simulink model "pmsm_foc"  (R2026a)
settings: Solver=ode4  StopTime=t_stop  FixedStep=P.Tsim
undefined symbols (not defined in the file or in its folder): P
settings Model: Creator=mask9  LastModifiedBy=mask9

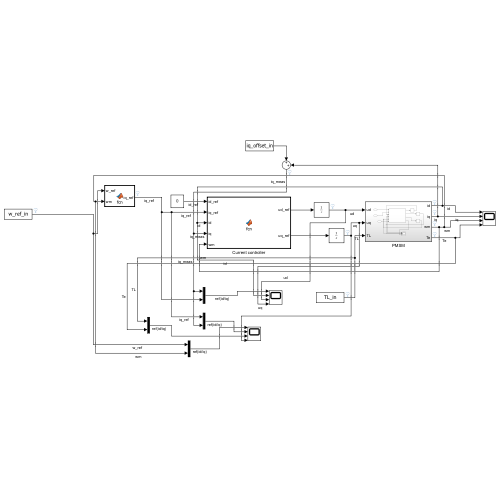
[thumbnail: Simulink's stored preview of the top-level diagram]
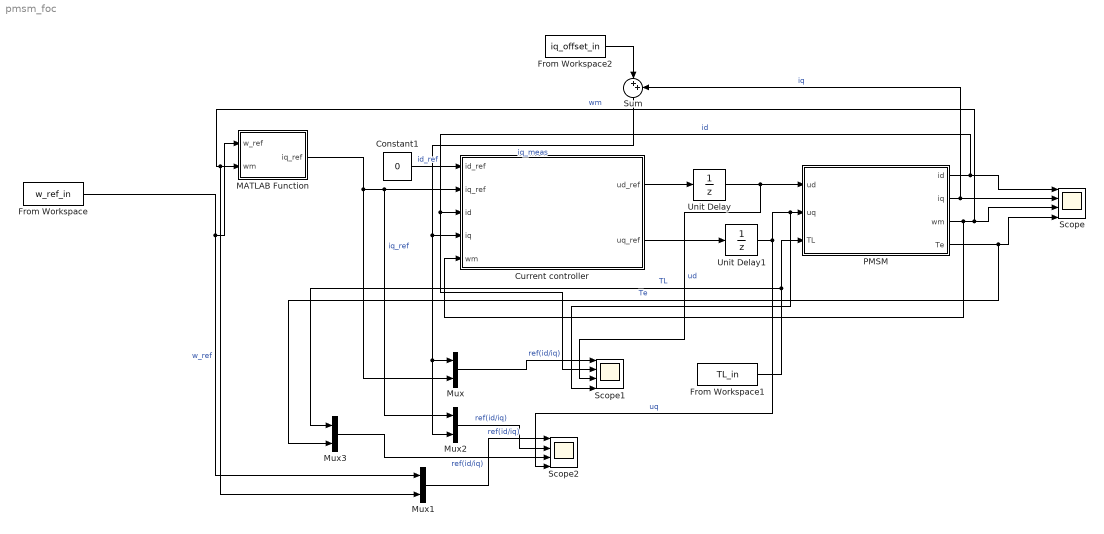
== system pmsm_foc ==
  Constant1 : Constant  Value=0
  Current controller : MATLAB Function  TreatAsAtomicUnit=on
  From Workspace : FromWorkspace  VariableName=w_ref_in  OutputAfterFinalValue=Holding final value
  From Workspace1 : FromWorkspace  VariableName=TL_in  OutputAfterFinalValue=Holding final value
  From Workspace2 : FromWorkspace  VariableName=iq_offset_in  OutputAfterFinalValue=Holding final value
  MATLAB Function : MATLAB Function  TreatAsAtomicUnit=on
  Mux{,1..3} (4 alike) : Mux  Inputs=2
  PMSM : Subsystem
  Scope : Scope  NumInputPorts=4
      settings: ActiveDisplayYMinimum=-7.6366046991371559E-6  ActiveDisplayYMaximum=6.8729442292234425E-5
  Scope1 : Scope  NumInputPorts=4
      settings: ActiveDisplayYMinimum=-60.523528989207882  ActiveDisplayYMaximum=544.71176090287111
  Scope2 : Scope  NumInputPorts=4
      settings: ActiveDisplayYMinimum=-6.2565775953438321  ActiveDisplayYMaximum=56.309198358094505  DataLoggingVariableName=ScopeData2
  Sum : Sum  Inputs=|++
  Unit Delay : UnitDelay  SampleTime=P.Ts
  Unit Delay1 : UnitDelay  SampleTime=P.Ts
  wires:
  From Workspace1/1 -> Mux3/1, PMSM/3(TL)  "TL"
  PMSM/1(id) -> Scope1/2, Current controller/3(id), Scope/1  "id"
  PMSM/2(iq) -> Sum/2, Scope/2  "iq"
  PMSM/3(wm) -> Current controller/5(wm), Mux1/2, MATLAB Function/2(wm), Scope/3  "wm"
  PMSM/4(Te) -> Mux3/2, Scope/4  "Te"
  Current controller/1(ud_ref) -> Unit Delay/1
  Unit Delay/1 -> Scope1/3, PMSM/1(ud)  "ud"
  Current controller/2(uq_ref) -> Unit Delay1/1
  Unit Delay1/1 -> Scope1/4, PMSM/2(uq), Scope2/4  "uq"
  Constant1/1 -> Current controller/1(id_ref)  "id_ref"
  Mux/1 -> Scope1/1  "ref(id/iq)"
  MATLAB Function/1(iq_ref) -> Mux/2, Mux2/1, Current controller/2(iq_ref)  "iq_ref"
  From Workspace/1 -> Mux1/1, MATLAB Function/1(w_ref)  "w_ref"
  Mux1/1 -> Scope2/1  "ref(id/iq)"
  Mux2/1 -> Scope2/2  "ref(id/iq)"
  Mux3/1 -> Scope2/3  "ref(id/iq)"
  From Workspace2/1 -> Sum/1
  Sum/1 -> Current controller/4(iq), Mux/1, Mux2/2  "iq_meas"

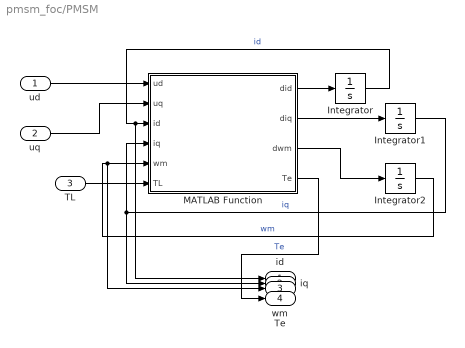
== system pmsm_foc/PMSM ==
  ud : Inport
  uq : Inport  Port=2
  TL : Inport  Port=3
  Integrator : Integrator
  Integrator1 : Integrator
  Integrator2 : Integrator
  MATLAB Function : MATLAB Function  TreatAsAtomicUnit=on
  id : Outport
  iq : Outport  Port=2
  wm : Outport  Port=3
  Te : Outport  Port=4
  wires:
  MATLAB Function/2(diq) -> Integrator1/1
  Integrator2/1 -> wm/1, MATLAB Function/5(wm)  "wm"
  MATLAB Function/3(dwm) -> Integrator2/1
  Integrator/1 -> id/1, MATLAB Function/3(id)  "id"
  uq/1 -> MATLAB Function/2(uq)
  Integrator1/1 -> iq/1, MATLAB Function/4(iq)  "iq"
  MATLAB Function/1(did) -> Integrator/1
  ud/1 -> MATLAB Function/1(ud)
  TL/1 -> MATLAB Function/6(TL)
  MATLAB Function/4(Te) -> Te/1  "Te"

== matlab function pmsm_foc/Current controller ==
  settings: updateMethod=DISCRETE  sampleTime=P.Ts
  data: id_ref input; ud_ref output; iq_ref input; id input; iq input; wm input; uq_ref output; P parameter
function [ud_ref, uq_ref] = fcn(id_ref, iq_ref, id, iq, wm, P)
persistent xd xq
if isempty(xd), xd = 0; xq = 0; end

we = P.p * wm;
ed = id_ref - id;
eq = iq_ref - iq;

% Decoupling feed-forward (cancels plant cross-coupling + back-EMF)
ud_ff = -we * P.Lq * iq;
uq_ff =  we * (P.Ld * id + P.psi);

% PI + feed-forward
ud_u = P.Kp_d*ed + xd + ud_ff;
uq_u = P.Kp_q*eq + xq + uq_ff;

% Voltage limit (circle, Umax = Udc/sqrt(3))
umag = sqrt(ud_u^2 + uq_u^2);
k = min(1, P.Umax / max(umag, 1e-9));
ud_ref = k * ud_u;
uq_ref = k * uq_u;

% Anti-windup: integrate only when not saturated
if k >= 1
    xd = xd + P.Ki_d * P.Ts * ed;
    xq = xq + P.Ki_q * P.Ts * eq;
end

== matlab function pmsm_foc/PMSM/MATLAB Function ==
  data: ud input; did output; uq input; id input; iq input; wm input; TL input; diq output; dwm output; Te output; P parameter
function [did, diq, dwm, Te] = fcn(ud, uq, id, iq, wm, TL, P)
we  = P.p * wm;
did = (ud - P.Rs*id + we*P.Lq*iq) / P.Ld;
diq = (uq - P.Rs*iq - we*P.Ld*id - we*P.psi) / P.Lq;
Te  = 1.5 * P.p * (P.psi*iq + (P.Ld - P.Lq)*id*iq);
dwm = (Te - TL - P.B*wm) / P.J;

== matlab function pmsm_foc/MATLAB Function ==
  settings: updateMethod=DISCRETE  sampleTime=P.Ts
  data: w_ref input; iq_ref output; wm input; P parameter
function iq_ref = fcn(w_ref, wm, P)
persistent xw
if isempty(xw), xw = 0; end

e = w_ref - wm;
u = P.Kp_w*e + xw;
iq_ref = min(max(u, -P.Imax), P.Imax);   % current limit 250 A

% Anti-windup: integrate only when not saturated
if iq_ref == u
    xw = xw + P.Ki_w*P.Ts*e;
end
